simulink model "ACC_konvoy"  (R2026a)
settings: Solver=ode4  StopTime=T_stop  FixedStep=dt
values from neighbouring files (symbols this model uses):
  d0 = 5    [ACC_yonetim.m]
  h = 1.2    [ACC_yonetim.m]
  Kd = 0.8    [ACC_yonetim.m]
  Kp = 0.4    [ACC_yonetim.m]
  L = 4.5    [ACC_yonetim.m]
  p0 = -(1:N) * (d_ss + L)    [ACC_yonetim.m]
  tau = 0.5    [ACC_yonetim.m]
  u_max = 3    [ACC_yonetim.m]
  u_min = -5    [ACC_yonetim.m]
  v0 = 15    [ACC_yonetim.m]
settings Model: Creator=furka  LastModifiedBy=furka

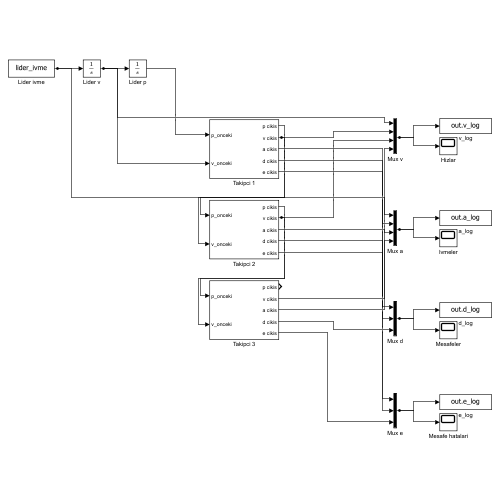
[thumbnail: Simulink's stored preview of the top-level diagram]
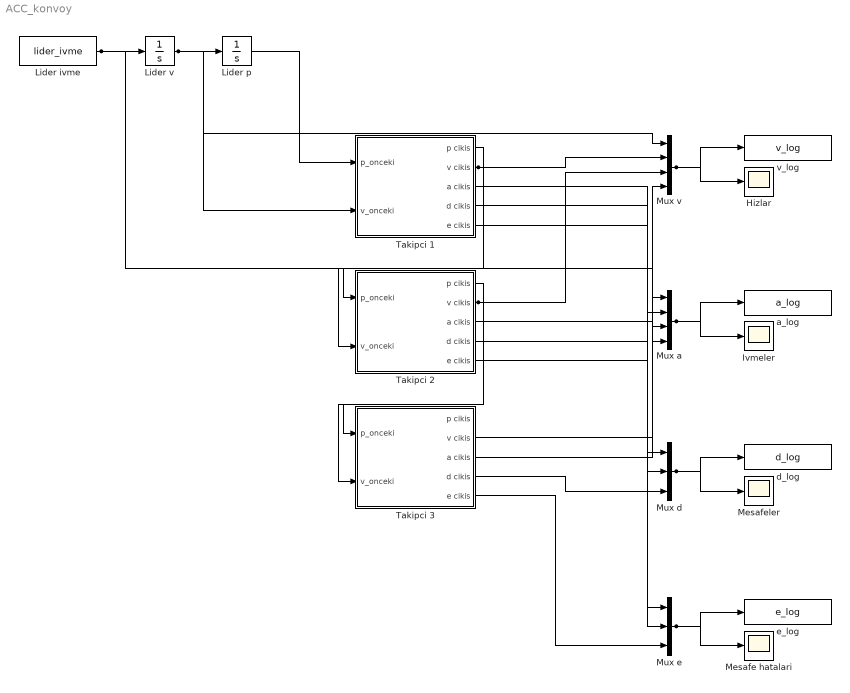
== system ACC_konvoy ==
  Hizlar : Scope
  Ivmeler : Scope
  Lider ivme : FromWorkspace  VariableName=lider_ivme  OutputAfterFinalValue=Holding final value
  Lider p : Integrator
  Lider v : Integrator  InitialCondition=v0
  Mesafe hatalari : Scope
  Mesafeler : Scope
  Mux a : Mux
  Mux d : Mux  Inputs=3
  Mux e : Mux  Inputs=3
  Mux v : Mux
  Takipci 1 : Subsystem
  Takipci 2 : Subsystem
  Takipci 3 : Subsystem
  a_log : ToWorkspace  VariableName=a_log  SampleTime=-1
  d_log : ToWorkspace  VariableName=d_log  SampleTime=-1
  e_log : ToWorkspace  VariableName=e_log  SampleTime=-1
  v_log : ToWorkspace  VariableName=v_log  SampleTime=-1
  wires:
  Lider ivme/1 -> Lider v/1, Mux a/1
  Lider v/1 -> Lider p/1, Takipci 1/2(v_onceki), Mux v/1
  Lider p/1 -> Takipci 1/1(p_onceki)
  Takipci 1/1(p cikis) -> Takipci 2/1(p_onceki)
  Takipci 1/2(v cikis) -> Takipci 2/2(v_onceki), Mux v/2
  Takipci 2/1(p cikis) -> Takipci 3/1(p_onceki)
  Takipci 2/2(v cikis) -> Takipci 3/2(v_onceki), Mux v/3
  Takipci 3/2(v cikis) -> Mux v/4
  Mux v/1 -> v_log/1, Hizlar/1
  Takipci 1/3(a cikis) -> Mux a/2
  Takipci 2/3(a cikis) -> Mux a/3
  Takipci 3/3(a cikis) -> Mux a/4
  Mux a/1 -> a_log/1, Ivmeler/1
  Takipci 1/4(d cikis) -> Mux d/1
  Takipci 2/4(d cikis) -> Mux d/2
  Takipci 3/4(d cikis) -> Mux d/3
  Mux d/1 -> d_log/1, Mesafeler/1
  Takipci 1/5(e cikis) -> Mux e/1
  Takipci 2/5(e cikis) -> Mux e/2
  Takipci 3/5(e cikis) -> Mux e/3
  Mux e/1 -> e_log/1, Mesafe hatalari/1

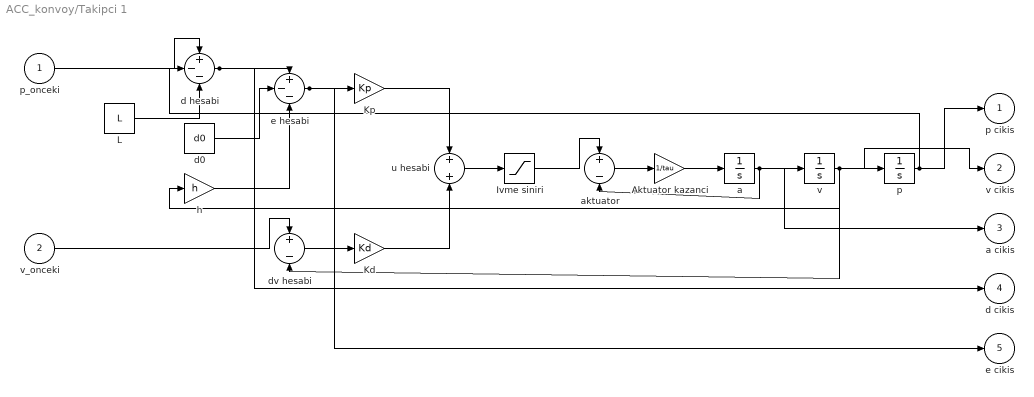
== system ACC_konvoy/Takipci 1 ==
  p_onceki : Inport
  v_onceki : Inport  Port=2
  Aktuator kazanci : Gain  Gain=1/tau
  Ivme siniri : Saturate  UpperLimit=u_max  LowerLimit=u_min
  Kd : Gain  Gain=Kd
  Kp : Gain  Gain=Kp
  L : Constant  Value=L
  a : Integrator
  aktuator : Sum  Inputs=+-
  d hesabi : Sum  Inputs=+--
  d0 : Constant  Value=d0
  dv hesabi : Sum  Inputs=+-
  e hesabi : Sum  Inputs=+--
  h : Gain  Gain=h
  p : Integrator  InitialCondition=p0(1)
  u hesabi : Sum
  v : Integrator  InitialCondition=v0
  p cikis : Outport
  v cikis : Outport  Port=2
  a cikis : Outport  Port=3
  d cikis : Outport  Port=4
  e cikis : Outport  Port=5
  wires:
  p_onceki/1 -> d hesabi/1
  p/1 -> d hesabi/2, p cikis/1
  L/1 -> d hesabi/3
  d hesabi/1 -> e hesabi/1, d cikis/1
  d0/1 -> e hesabi/2
  v/1 -> h/1, dv hesabi/2, p/1, v cikis/1
  h/1 -> e hesabi/3
  v_onceki/1 -> dv hesabi/1
  e hesabi/1 -> Kp/1, e cikis/1
  dv hesabi/1 -> Kd/1
  Kp/1 -> u hesabi/1
  Kd/1 -> u hesabi/2
  u hesabi/1 -> Ivme siniri/1
  Ivme siniri/1 -> aktuator/1
  a/1 -> aktuator/2, v/1, a cikis/1
  aktuator/1 -> Aktuator kazanci/1
  Aktuator kazanci/1 -> a/1

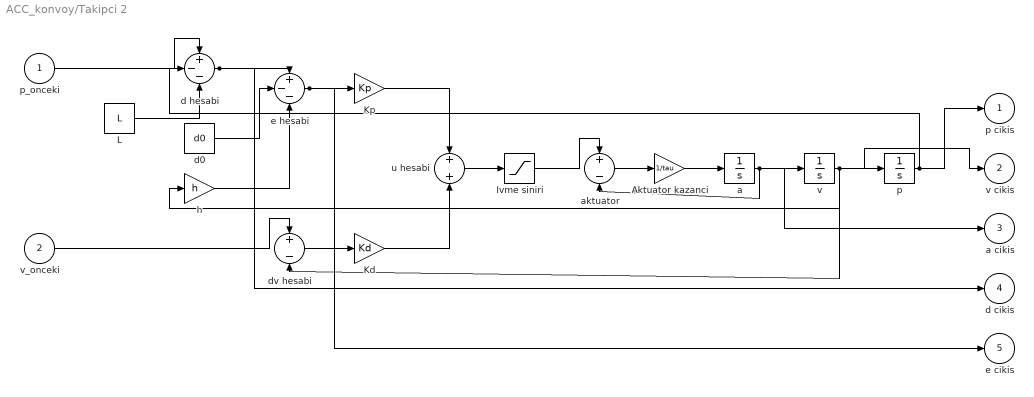
== system ACC_konvoy/Takipci 2 ==
  p_onceki : Inport
  v_onceki : Inport  Port=2
  Aktuator kazanci : Gain  Gain=1/tau
  Ivme siniri : Saturate  UpperLimit=u_max  LowerLimit=u_min
  Kd : Gain  Gain=Kd
  Kp : Gain  Gain=Kp
  L : Constant  Value=L
  a : Integrator
  aktuator : Sum  Inputs=+-
  d hesabi : Sum  Inputs=+--
  d0 : Constant  Value=d0
  dv hesabi : Sum  Inputs=+-
  e hesabi : Sum  Inputs=+--
  h : Gain  Gain=h
  p : Integrator  InitialCondition=p0(2)
  u hesabi : Sum
  v : Integrator  InitialCondition=v0
  p cikis : Outport
  v cikis : Outport  Port=2
  a cikis : Outport  Port=3
  d cikis : Outport  Port=4
  e cikis : Outport  Port=5
  wires:
  p_onceki/1 -> d hesabi/1
  p/1 -> d hesabi/2, p cikis/1
  L/1 -> d hesabi/3
  d hesabi/1 -> e hesabi/1, d cikis/1
  d0/1 -> e hesabi/2
  v/1 -> h/1, dv hesabi/2, p/1, v cikis/1
  h/1 -> e hesabi/3
  v_onceki/1 -> dv hesabi/1
  e hesabi/1 -> Kp/1, e cikis/1
  dv hesabi/1 -> Kd/1
  Kp/1 -> u hesabi/1
  Kd/1 -> u hesabi/2
  u hesabi/1 -> Ivme siniri/1
  Ivme siniri/1 -> aktuator/1
  a/1 -> aktuator/2, v/1, a cikis/1
  aktuator/1 -> Aktuator kazanci/1
  Aktuator kazanci/1 -> a/1

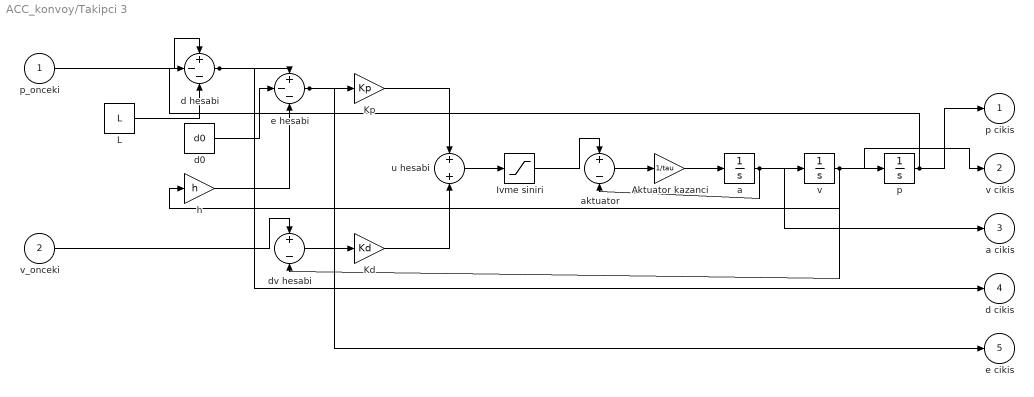
== system ACC_konvoy/Takipci 3 ==
  p_onceki : Inport
  v_onceki : Inport  Port=2
  Aktuator kazanci : Gain  Gain=1/tau
  Ivme siniri : Saturate  UpperLimit=u_max  LowerLimit=u_min
  Kd : Gain  Gain=Kd
  Kp : Gain  Gain=Kp
  L : Constant  Value=L
  a : Integrator
  aktuator : Sum  Inputs=+-
  d hesabi : Sum  Inputs=+--
  d0 : Constant  Value=d0
  dv hesabi : Sum  Inputs=+-
  e hesabi : Sum  Inputs=+--
  h : Gain  Gain=h
  p : Integrator  InitialCondition=p0(3)
  u hesabi : Sum
  v : Integrator  InitialCondition=v0
  p cikis : Outport
  v cikis : Outport  Port=2
  a cikis : Outport  Port=3
  d cikis : Outport  Port=4
  e cikis : Outport  Port=5
  wires:
  p_onceki/1 -> d hesabi/1
  p/1 -> d hesabi/2, p cikis/1
  L/1 -> d hesabi/3
  d hesabi/1 -> e hesabi/1, d cikis/1
  d0/1 -> e hesabi/2
  v/1 -> h/1, dv hesabi/2, p/1, v cikis/1
  h/1 -> e hesabi/3
  v_onceki/1 -> dv hesabi/1
  e hesabi/1 -> Kp/1, e cikis/1
  dv hesabi/1 -> Kd/1
  Kp/1 -> u hesabi/1
  Kd/1 -> u hesabi/2
  u hesabi/1 -> Ivme siniri/1
  Ivme siniri/1 -> aktuator/1
  a/1 -> aktuator/2, v/1, a cikis/1
  aktuator/1 -> Aktuator kazanci/1
  Aktuator kazanci/1 -> a/1
